simulink model "FAST_11TO14mpers_MPC"  (R2019a)
settings: Solver=FixedStepAuto  StartTime=0.0  StopTime=10  FixedStep=DT  RelTol=1e-3
values from neighbouring files (symbols this model uses):
  Cq = 0.0 0.0 0.0 0.0 0.0 0.0 0.0 0.0 0.0 0.0 0.0 0.0 0.0 0.0 0.0 0.0 0.0 0.0 0.0 0.0 0.0 0.0 0.0 0.0 0.0 0.0 0.0 0.0 0.0 0.0 0.0 0.0 0.0 0.0 0.0 0.0 0.0 0.0 0.0 0.0 0.0 0.0 0.0 0.0 0.0 0.0 0.0 0.0 0.0 0.0 0.0 0.0 0.0 0.0 0.0 0.0 0.0 0.0 0.0 0.0 0.0 0.0 0.0 0.0 0.0 0.0 0.0 0.0 0.0 0.0 0.0 0.0 0.0 0.0 0.0 0.0 0.0 0.0 0.0 0.0 0.0 0.0 0.0 0.0 0.0 0.0 0.0 0.0 0.0 0.0 0.0 0.0 0.0 0.0 0.0 0.0 0.0 0.0 0.0 0.0    [DD_test.sldd]    (also in testOutList.m = saveVarsMat.Cq)
  Drivetrain = struct    [dataDLR.m]
  DT = 0.008    [dataDLR.m]    (also in generateReport.m; initLPVParam.m; initWorkspace.m; runCalculateEvalCriteria.m)
  Lin_points : value not decoded    [DD_test.sldd]
  mu_old = zeros(2*N*nu,1)    [testCtrl.m]
  Ng = 97    [dataDLR.m]    (also in testCtrl.m)
  omegabar = interp1(Lin_points.V,Lin_points.RSpeed,Vbar,'spline')    [testCtrl.m]
  OutList = OutTable.Properties.VariableNames    [initLPVParam.m]    (also in testCtrl.m; testOutList.m = cell(40, 1); testqLPV.m = cell(40, 1))
  tau_g = 0.01    [testCtrl.m]
  U = zeros(2*N,1)    [testCtrl.m]
  Xk07 = kron(ones(N,1),xk07)    [testCtrl.m]
  xk07 = [r7(1), r7(2), zeros(1,5),0]'    [testCtrl.m]
undefined symbols (not defined in the file or in its folder): Rotor_Lambda, Rotor_Lamda, Rotor_Pitch, strmatch
libraries: MdlLib_ProcessOutput x1
settings Model: ExtModeTrigMode=oneshot  ExtModeArmWhenConnect=off  Creator=Hazim Namik  LastModifiedBy=ditt_aj
settings DataIOCC: LimitDataPoints=on  SaveFormat=Array  ReturnWorkspaceOutputs=off
settings OptimizationCC: BlockReduction=off  BooleanDataType=off  LifeSpan=inf
settings DebuggingCC: SaveWithParameterizedLinksMsg=none  UnderspecifiedInitializationDetection=Classic  MergeDetectMultiDrivingBlocksExec=none  SignalResolutionControl=TryResolveAllWithWarning  SFUnexpectedBacktrackingDiag=warning  SFNoUnconditionalDefaultTransitionDiag=warning  SFExecutionAtInitializationDiag=none  ArithmeticOperatorsInVariantConditions=warning
settings HardwareCC: ProdBitPerPointer=32  ProdBitPerSizeT=32  ProdBitPerPtrDiffT=32  ProdLargestAtomicFloat=None  ProdIntDivRoundTo=Undefined  ProdEndianess=Unspecified  ProdWordSize=32  ProdHWDeviceType=32-bit Generic  TargetUnknown=on
settings ModelReferenceCC: PropagateSignalLabelsOutOfModel=off
settings SFSimCC: SimUseLocalCustomCode=off
settings RTWCC: RTWUseLocalCustomCode=off
settings CodeAppCC: StateflowObjectComments=on
settings GRTTargetCC: TargetLangStandard=C89/C90 (ANSI)  GeneratePreprocessorConditionals=Disable all
settings ConfigComp: CovMetricSettings=dw  CovHtmlReporting=on  CovSaveCumulativeToWorkspaceVar=on  CovSaveSingleToWorkspaceVar=on  CovExternalEMLEnable=off

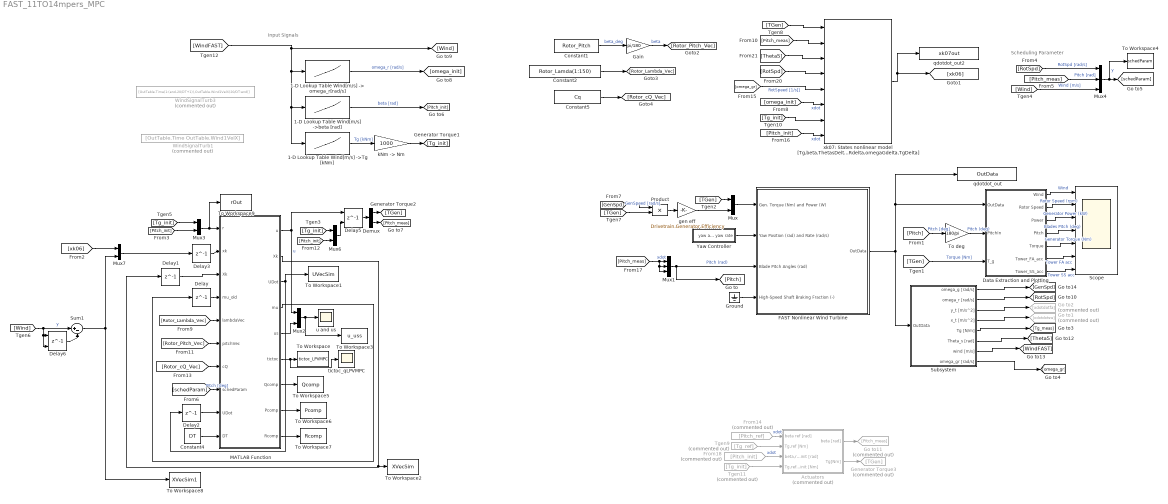
== system FAST_11TO14mpers_MPC ==
  note: Scheduling Parameter
  note: Input Signals
  "1-D Lookup Table Wind[m/s] -> omega_r[rad/s]" : Lookup_n-D  NumberOfTableDimensions=1  BreakpointsForDimension1=Lin_points.V  BreakpointsForDimension2=Rotor_Lambda  Table=Lin_points.RSpeed  InternalRulePriority=Speed  RndMeth=Simplest  InputSameDT=on
  1-D Lookup Table Wind[m/s] ->Tg [kNm] : Lookup_n-D  NumberOfTableDimensions=1  BreakpointsForDimension1=Lin_points.V  BreakpointsForDimension2=Rotor_Lambda  Table=Lin_points.Torque  InternalRulePriority=Speed  RndMeth=Simplest  InputSameDT=on
  1-D Lookup Table Wind[m/s] ->beta [rad] : Lookup_n-D  NumberOfTableDimensions=1  BreakpointsForDimension1=Lin_points.V  BreakpointsForDimension2=Rotor_Lambda  Table=Lin_points.Pitch  InternalRulePriority=Speed  RndMeth=Simplest  InputSameDT=on
  Actuators : Subsystem  Commented=on
  Constant1 : Constant  Value=Rotor_Pitch
  Constant2 : Constant  Value=Rotor_Lamda(1:150)
  Constant4 : Constant  Value=DT
  Constant5 : Constant  Value=Cq
  Data Extraction and Plotting : Subsystem
  Delay : Delay  DelayLength=1  InitialCondition=mu_old
  Delay1 : Delay  DelayLength=1  InitialCondition=Xk07
  Delay2 : Delay  DelayLength=1  InitialCondition=U
  Delay3 : Delay  DelayLength=1  InitialCondition=xk07
  Delay5 : Delay  DelayLength=1  InitialConditionSource=Input port  InitialCondition=[0,omegabar]
      settings: InputPortMap=u0,p4
  Delay6 : Delay  DelayLength=1  InitialConditionSource=Input port  InitialCondition=[0, Lin_points.Torque(1)]
      settings: InputPortMap=u0,p4
  Demux : Demux  Outputs=2
  FAST Nonlinear Wind Turbine : Subsystem  mask(FAST Nonlinear Wind Turbine){}
      mask help: This block contains the FAST S-Function.
      mask init:
      | clear FAST_SFunc
  From14 : From  Commented=on  GotoTag=Pitch_ref
      settings: CloseFcn=tagdialog Close
  From18 : From  Commented=on  GotoTag=Pitch_init
      settings: CloseFcn=tagdialog Close
  Gain : Gain  Gain=pi/180
  Generator Torque3 : Goto  Commented=on  GotoTag=TGen
  Go to1 : Goto  Commented=on  GotoTag=xdotdotsw
  Go to11 : Goto  Commented=on  GotoTag=Pitch_meas
  Go to2 : Goto  Commented=on  GotoTag=xdotdotfa
  Ground : Ground
  MATLAB Function : MATLAB Function  TreatAsAtomicUnit=on
  Mux{,2..3,6..7} (5 alike) : Mux  Inputs=2
  Mux1 : Mux  Inputs=3
  Mux4 : Mux  Inputs=3
  Product : Product  RndMeth=Zero
  Scope : Scope  NumInputPorts=7
      settings: Tag=Scope
  Subsystem : Subsystem
  Sum1 : Sum  Inputs=|+-
  Tgen11 : From  Commented=on  GotoTag=Tg_init
      settings: CloseFcn=tagdialog Close
  Tgen9 : From  Commented=on  GotoTag=Tg_ref
      settings: CloseFcn=tagdialog Close
  To Workspace : ToWorkspace  VariableName=tictoc_LPVMPC  SaveFormat=Timeseries  SampleTime=-1
  To Workspace1 : ToWorkspace  VariableName=UVecSim  SampleTime=-1
  To Workspace2 : ToWorkspace  VariableName=XVecSim  SampleTime=-1
  To Workspace3 : ToWorkspace  VariableName=u_uss  SampleTime=-1
      settings: Save2DSignal=2-D array (concatenate along first dimension)
  To Workspace4 : ToWorkspace  VariableName=schedParam  SampleTime=-1
      settings: Save2DSignal=2-D array (concatenate along first dimension)
  To Workspace5 : ToWorkspace  VariableName=Qcomp  SampleTime=-1
      settings: Save2DSignal=2-D array (concatenate along first dimension)
  To Workspace6 : ToWorkspace  VariableName=Pcomp  SampleTime=-1
      settings: Save2DSignal=2-D array (concatenate along first dimension)
  To Workspace7 : ToWorkspace  VariableName=Rcomp  SampleTime=-1
      settings: Save2DSignal=2-D array (concatenate along first dimension)
  To Workspace8 : ToWorkspace  VariableName=XVecSim1  SampleTime=-1
  To Workspace9 : ToWorkspace  VariableName=rOut  SampleTime=-1
  To deg : Gain  Gain=180/pi
  WindSignalTurb1 : FromWorkspace  Commented=on  VariableName=[OutTable.Time OutTable.Wind1VelX]  SampleTime=DT  OutputAfterFinalValue=Holding final value
  WindSignalTurb3 : FromWorkspace  Commented=on  VariableName=[OutTable.Time(1:(end-20/DT+1)),OutTable.Wind1VelX(20/DT:end)]  SampleTime=DT  OutputAfterFinalValue=Holding final value
  Yaw Controller : Subsystem
  gen eff : Gain  Gain=Drivetrain.Generator.Efficiency
  "kNm -> Nm" : Gain  Gain=1000
  qdotdot_out : ToWorkspace  VariableName=OutData  SampleTime=-1
  qdotdot_out2 : ToWorkspace  VariableName=xk07out  SampleTime=-1
  tictoc_qLPVMPC : Scope
  u and us : Scope
  xk07: States nonlinear model [Tg,beta,ThetasDelta,omegaRdelta,omegaGdelta,TgDelta] : MdlLib_ProcessOutput/xk07: States nonlinear model [Tg,beta,ThetasDelta,omegaRdelta,omegaGdelta,TgDelta]  SystemSampleTime=-1
  wires:
  Mux/1 -> FAST Nonlinear Wind Turbine/1(Gen. Torque (Nm) and Power (W))
  Yaw Controller/1(yaw and yaw rate) -> FAST Nonlinear Wind Turbine/2(Yaw Position (rad) and Rate (rad/s))
  Mux1/1 -> [Pitch], FAST Nonlinear Wind Turbine/3(Blade Pitch Angles (rad))  "Pitch (rad)"
  gen eff/1 -> Mux/2
  Product/1 -> gen eff/1
  Data Extraction and Plotting/3(Power) -> Scope/3  "Generator Power (kW)"
  [Pitch] -> To deg/1  "Pitch [deg]"
  Data Extraction and Plotting/1(Wind) -> Scope/1  "Wind"
  Data Extraction and Plotting/2(Rotor Speed) -> Scope/2  "Rotor Speed (rpm)"
  [TGen] -> Data Extraction and Plotting/3(T_g)  "Torque [Nm]"
  FAST Nonlinear Wind Turbine/1(OutData) -> Subsystem/1(OutData), qdotdot_out/1, Data Extraction and Plotting/1(OutData)
  Data Extraction and Plotting/4(Pitch) -> Scope/4  "Blades Pitch (deg)"
  Data Extraction and Plotting/5(Torque) -> Scope/5  "Generator Torque (Nm)"
  Data Extraction and Plotting/6(Tower_FA_acc) -> Scope/6  "Tower FA acc"
  Data Extraction and Plotting/7(Tower_SS_acc) -> Scope/7  "Tower SS acc"
  Ground/1 -> FAST Nonlinear Wind Turbine/4(High-Speed Shaft Braking Fraction (-))
  [TGen] -> Mux/1
  Subsystem/8(omega_gr [rad/s]) -> [omega_gr]
  Subsystem/3(y_t [m/s^2]) -> Go to2/1
  Subsystem/4(x_t [m/s^2]) -> Go to1/1
  Subsystem/5(Tg [N/m]) -> [Tg_meas]
  [GenSpd] -> Product/1  "GenSpeed [rad/s]"
  [Pitch_meas] -> Mux4/2  "Pitch [rad]"
  [Tg_init] -> xk07: States nonlinear model [Tg,beta,ThetasDelta,omegaRdelta,omegaGdelta,TgDelta]/7
  [Wind] -> Mux4/3  "Wind [m/s]"
  [Pitch_meas] -> xk07: States nonlinear model [Tg,beta,ThetasDelta,omegaRdelta,omegaGdelta,TgDelta]/2
  [RotSpd] -> Mux4/1  "RotSpd [rad/s]"
  [omega_init] -> xk07: States nonlinear model [Tg,beta,ThetasDelta,omegaRdelta,omegaGdelta,TgDelta]/6  "xdot"
  [Pitch_init] -> xk07: States nonlinear model [Tg,beta,ThetasDelta,omegaRdelta,omegaGdelta,TgDelta]/8  "xdot"
  [TGen] -> xk07: States nonlinear model [Tg,beta,ThetasDelta,omegaRdelta,omegaGdelta,TgDelta]/1
  Constant5/1 -> [Rotor_cQ_Vec]
  xk07: States nonlinear model [Tg,beta,ThetasDelta,omegaRdelta,omegaGdelta,TgDelta]/1 -> [xk06], qdotdot_out2/1
  [omega_gr] -> xk07: States nonlinear model [Tg,beta,ThetasDelta,omegaRdelta,omegaGdelta,TgDelta]/5  "RotSpeed [1/s]]"
  [ThetaS] -> xk07: States nonlinear model [Tg,beta,ThetasDelta,omegaRdelta,omegaGdelta,TgDelta]/3
  [RotSpd] -> xk07: States nonlinear model [Tg,beta,ThetasDelta,omegaRdelta,omegaGdelta,TgDelta]/4
  Gain/1 -> [Rotor_Pitch_Vec]  "beta"
  Constant1/1 -> Gain/1  "beta_deg"
  Mux4/1 -> To Workspace4/1, [schedParam]  "y"
  Constant2/1 -> [Rotor_Lambda_Vec]
  [WindFAST] -> "1-D Lookup Table Wind[m/s] -> omega_r[rad/s]"/1, 1-D Lookup Table Wind[m/s] ->beta [rad]/1, 1-D Lookup Table Wind[m/s] ->Tg [kNm]/1, [Wind]
  "1-D Lookup Table Wind[m/s] -> omega_r[rad/s]"/1 -> [omega_init]  "omega_r [rad/s]"
  1-D Lookup Table Wind[m/s] ->Tg [kNm]/1 -> "kNm -> Nm"/1  "Tg [kNm]"
  "kNm -> Nm"/1 -> [Tg_init]
  1-D Lookup Table Wind[m/s] ->beta [rad]/1 -> [Pitch_init]  "beta [rad]"
  Demux/1 -> [TGen]
  MATLAB Function/3(UDot) -> Delay2/1, To Workspace1/1
  Delay6/1 -> Sum1/2
  Delay3/1 -> MATLAB Function/2(xk)
  Delay2/1 -> MATLAB Function/9("UDot ")
  Mux2/1 -> u and us/1, To Workspace3/1
  [Rotor_Lambda_Vec] -> MATLAB Function/5(lambdaVec)
  [Tg_init] -> Mux3/1
  MATLAB Function/7(Qcomp) -> To Workspace5/1
  Constant4/1 -> MATLAB Function/10(DT)
  [Tg_init] -> Mux6/1
  [Pitch_init] -> Mux6/2
  [schedParam] -> MATLAB Function/8(schedParam)  "Pitch [deg]"
  Delay5/1 -> Demux/1
  Mux7/1 -> Delay3/1
  Demux/2 -> [Pitch_meas]
  Mux6/1 -> Delay5/2
  [Wind] -> Delay6/2, Delay6/1, Sum1/1  "y"
  [xk06] -> Mux7/1
  [Rotor_cQ_Vec] -> MATLAB Function/7(cQ)
  Sum1/1 -> To Workspace8/1, Mux7/2
  MATLAB Function/8(Pcomp) -> To Workspace6/1
  MATLAB Function/9(Rcomp) -> To Workspace7/1
  [Rotor_Pitch_Vec] -> MATLAB Function/6(pitchVec)
  Mux3/1 -> To Workspace9/1, MATLAB Function/1(r)
  MATLAB Function/1(u) -> Delay5/1, Mux2/1  "u"
  Delay1/1 -> MATLAB Function/3("Xk ")
  [Pitch_init] -> Mux3/2
  Delay/1 -> MATLAB Function/4(mu_old)
  MATLAB Function/6(tictoc) -> tictoc_qLPVMPC/1, To Workspace/1
  MATLAB Function/2(Xk) -> Delay1/1, To Workspace2/1
  MATLAB Function/4(mu) -> Delay/1
  MATLAB Function/5(us) -> Mux2/2
  [Pitch_meas] -> Mux1/3, Mux1/2, Mux1/1  "xdot"
  Subsystem/2(omega_r [rad/s]) -> [RotSpd]
  Actuators/2(Tg[Nm]) -> Generator Torque3/1
  Tgen9/1 -> Actuators/2(Tg,ref [Nm])
  From14/1 -> Actuators/1(beta ref [rad])  "xdot"
  Actuators/1(beta [rad]) -> Go to11/1
  [TGen] -> Product/2
  Tgen11/1 -> Actuators/4(Tg,ref init [Nm])
  From18/1 -> Actuators/3(beta,ref init [rad])  "xdot"
  Subsystem/6(Theta_s [rad]) -> [ThetaS]
  Subsystem/7(wind [m/s]) -> [WindFAST]
  Subsystem/1(omega_g [rad/s]) -> [GenSpd]
  To deg/1 -> Data Extraction and Plotting/2(PitchIn)  "Pitch (deg)"

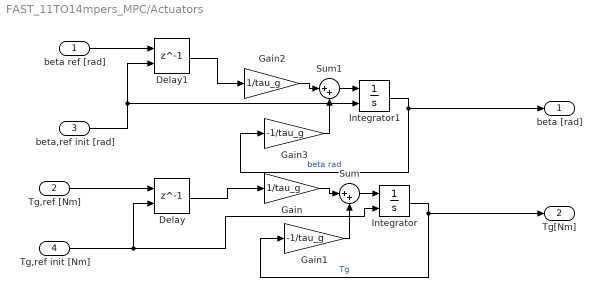
== system FAST_11TO14mpers_MPC/Actuators ==
  beta ref [rad] : Inport
  Tg,ref [Nm] : Inport  Port=2
  beta,ref init [rad] : Inport  Port=3
  Tg,ref init [Nm] : Inport  Port=4
  Delay : Delay  DelayLength=1  InitialConditionSource=Input port
      settings: InputPortMap=u0,p4
  Delay1 : Delay  DelayLength=1  InitialConditionSource=Input port
      settings: InputPortMap=u0,p4
  Gain : Gain  Gain=1/tau_g
  Gain1 : Gain  Gain=-1/tau_g
  Gain2 : Gain  Gain=1/tau_g
  Gain3 : Gain  Gain=-1/tau_g
  Integrator : Integrator  InitialConditionSource=external
  Integrator1 : Integrator  InitialConditionSource=external
  Sum : Sum  Inputs=|++
  Sum1 : Sum  Inputs=|++
  beta [rad] : Outport
  Tg[Nm] : Outport  Port=2
  wires:
  Sum1/1 -> Integrator1/1
  Integrator/1 -> Tg[Nm]/1, Gain1/1  "Tg"
  Tg,ref init [Nm]/1 -> Delay/2, Integrator/2
  Gain3/1 -> Sum1/2
  Gain2/1 -> Sum1/1
  Sum/1 -> Integrator/1
  Gain1/1 -> Sum/2
  Integrator1/1 -> beta [rad]/1, Gain3/1  "beta rad"
  Gain/1 -> Sum/1
  Tg,ref [Nm]/1 -> Delay/1
  Delay/1 -> Gain/1
  beta ref [rad]/1 -> Delay1/1
  Delay1/1 -> Gain2/1
  beta,ref init [rad]/1 -> Integrator1/2, Delay1/2

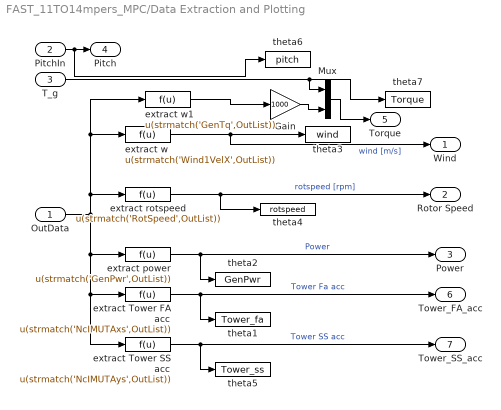
== system FAST_11TO14mpers_MPC/Data Extraction and Plotting ==
  OutData : Inport
  PitchIn : Inport  Port=2
  T_g : Inport  Port=3
  Gain : Gain  Gain=1000
  Mux : Mux  Inputs=2
  extract Tower FA acc : Fcn  Expr=u(strmatch('NcIMUTAxs',OutList))
  extract Tower SS acc : Fcn  Expr=u(strmatch('NcIMUTAys',OutList))
  extract power : Fcn  Expr=u(strmatch('GenPwr',OutList))
  extract rotspeed : Fcn  Expr=u(strmatch('RotSpeed',OutList))
  extract w : Fcn  Expr=u(strmatch('Wind1VelX',OutList))
  extract w1 : Fcn  Expr=u(strmatch('GenTq',OutList))
  theta1 : ToWorkspace  VariableName=Tower_fa  SampleTime=-1
      settings: MaxDataPoints=Inf  Decimation=3
  theta2 : ToWorkspace  VariableName=GenPwr  SampleTime=-1
      settings: MaxDataPoints=Inf  Decimation=3
  theta3 : ToWorkspace  VariableName=wind  SampleTime=-1
      settings: MaxDataPoints=Inf  Decimation=3
  theta4 : ToWorkspace  VariableName=rotspeed  SampleTime=-1
      settings: MaxDataPoints=Inf  Decimation=3
  theta5 : ToWorkspace  VariableName=Tower_ss  SampleTime=-1
      settings: MaxDataPoints=Inf  Decimation=3
  theta6 : ToWorkspace  VariableName=pitch  SampleTime=-1
      settings: MaxDataPoints=Inf  Decimation=3
  theta7 : ToWorkspace  VariableName=Torque  SampleTime=-1
      settings: MaxDataPoints=Inf  Decimation=3
  Wind : Outport
  Rotor Speed : Outport  Port=2
  Power : Outport  Port=3
  Pitch : Outport  Port=4
  Torque : Outport  Port=5
  Tower_FA_acc : Outport  Port=6
  Tower_SS_acc : Outport  Port=7
  wires:
  extract w/1 -> Wind/1, theta3/1  "wind [m/s]"
  extract rotspeed/1 -> theta4/1, Rotor Speed/1  "rotspeed [rpm]"
  extract power/1 -> theta2/1, Power/1  "Power"
  PitchIn/1 -> theta6/1, Pitch/1
  T_g/1 -> Mux/1, theta7/1
  extract Tower FA acc/1 -> theta1/1, Tower_FA_acc/1  "Tower Fa acc"
  OutData/1 -> extract w/1, extract w1/1, extract rotspeed/1, extract Tower SS acc/1, extract Tower FA acc/1, extract power/1
  extract Tower SS acc/1 -> theta5/1, Tower_SS_acc/1  "Tower SS acc"
  extract w1/1 -> Gain/1
  Gain/1 -> Mux/2
  Mux/1 -> Torque/1

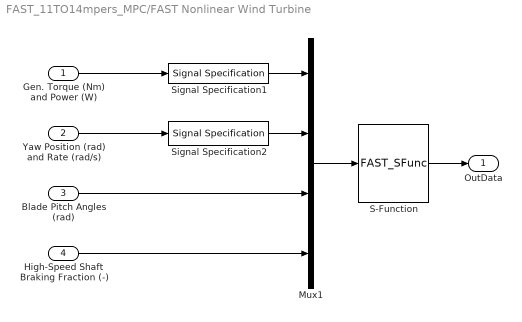
== system FAST_11TO14mpers_MPC/FAST Nonlinear Wind Turbine ==
  Gen. Torque (Nm) and Power (W) : Inport
  Yaw Position (rad) and Rate (rad/s) : Inport  Port=2
  Blade Pitch Angles (rad) : Inport  Port=3
  High-Speed Shaft Braking Fraction (-) : Inport  Port=4
  Mux1 : Mux
  S-Function : S-Function  FunctionName=FAST_SFunc  Parameters=FAST_InputFileName, TMax, 0  SFunctionDeploymentMode=off  EnableBusSupport=off
  Signal Specification1 : SignalSpecification  OutDataTypeStr=double  Dimensions=2
  Signal Specification2 : SignalSpecification  OutDataTypeStr=double  Dimensions=2
  OutData : Outport
  wires:
  Gen. Torque (Nm) and Power (W)/1 -> Signal Specification1/1
  S-Function/1 -> OutData/1
  Mux1/1 -> S-Function/1
  Blade Pitch Angles (rad)/1 -> Mux1/3
  Yaw Position (rad) and Rate (rad/s)/1 -> Signal Specification2/1
  Signal Specification1/1 -> Mux1/1
  Signal Specification2/1 -> Mux1/2
  High-Speed Shaft Braking Fraction (-)/1 -> Mux1/4

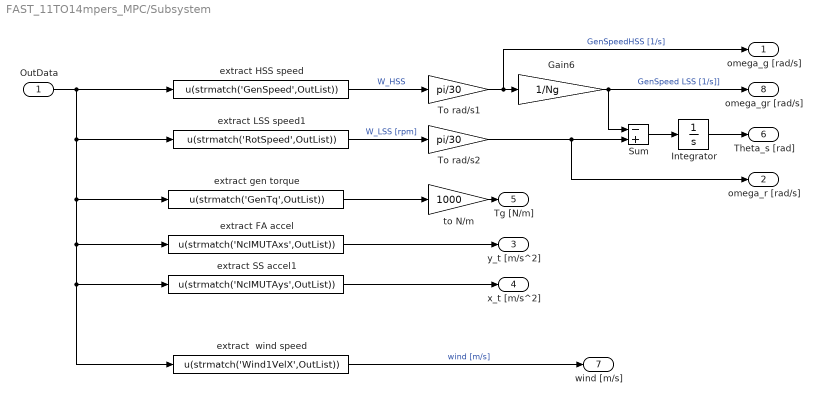
== system FAST_11TO14mpers_MPC/Subsystem ==
  OutData : Inport
  Gain6 : Gain  Gain=1/Ng
  Integrator : Integrator
  Sum : Sum  Inputs=-+
  To rad/s1 : Gain  Gain=pi/30
  To rad/s2 : Gain  Gain=pi/30
  extract  wind speed : Fcn  Expr=u(strmatch('Wind1VelX',OutList))
  extract FA accel : Fcn  Expr=u(strmatch('NcIMUTAxs',OutList))
  extract HSS speed : Fcn  Expr=u(strmatch('GenSpeed',OutList))
  extract LSS speed1 : Fcn  Expr=u(strmatch('RotSpeed',OutList))
  extract SS accel1 : Fcn  Expr=u(strmatch('NcIMUTAys',OutList))
  extract gen torque : Fcn  Expr=u(strmatch('GenTq',OutList))
  to N/m : Gain  Gain=1000
  omega_g [rad/s] : Outport
  omega_r [rad/s] : Outport  Port=2
  y_t [m/s^2] : Outport  Port=3
  x_t [m/s^2] : Outport  Port=4
  Tg [N/m] : Outport  Port=5
  Theta_s [rad] : Outport  Port=6
  wind [m/s] : Outport  Port=7
  omega_gr [rad/s] : Outport  Port=8
  wires:
  to N/m/1 -> Tg [N/m]/1
  OutData/1 -> extract HSS speed/1, extract  wind speed/1, extract SS accel1/1, extract FA accel/1, extract gen torque/1, extract LSS speed1/1
  extract FA accel/1 -> y_t [m/s^2]/1
  extract HSS speed/1 -> To rad/s1/1  "W_HSS"
  extract gen torque/1 -> to N/m/1
  extract SS accel1/1 -> x_t [m/s^2]/1
  To rad/s1/1 -> omega_g [rad/s]/1, Gain6/1  "GenSpeedHSS [1/s]"
  extract LSS speed1/1 -> To rad/s2/1  "W_LSS [rpm]"
  Gain6/1 -> Sum/1, omega_gr [rad/s]/1  "GenSpeed LSS [1/s]]"
  To rad/s2/1 -> Sum/2, omega_r [rad/s]/1
  Sum/1 -> Integrator/1
  Integrator/1 -> Theta_s [rad]/1
  extract  wind speed/1 -> wind [m/s]/1  "wind [m/s]"

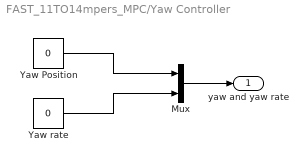
== system FAST_11TO14mpers_MPC/Yaw Controller ==
  Mux : Mux  Inputs=2
  Yaw Position : Constant  Value=0
  Yaw rate : Constant  Value=0
  yaw and yaw rate : Outport
  wires:
  Mux/1 -> yaw and yaw rate/1
  Yaw Position/1 -> Mux/1
  Yaw rate/1 -> Mux/2

== matlab function FAST_11TO14mpers_MPC/MATLAB Function ==
  settings: updateMethod=DISCRETE
  data: r input; u output; xk input; Xk input; mu_old input; lambdaVec input; pitchVec input; cQ input; schedParam input; UDot input; DT input; Xk output; UDot output; mu output; us output; tictoc output; Qcomp output; Pcomp output; Rcomp output
function [u,Xk,UDot,mu,us,tictoc, Qcomp,Pcomp,Rcomp]= qLPVMPC_WECS_beta(r,xk,Xk,mu_old,lambdaVec,pitchVec,cQ,schedParam,UDot,DT)
% MATLAB_Function calculates controller output u. It turns the QP into a 
% linear complementarity problem (LCP) and solves it with Lemke's algorithm.
%
% Inputs: * r: reference
%         * xk: quasiLPV KF state estimates
%         * Xk: Xko(= L*xk+S*U) delayed by one sample timestep
%         * mu_old: mu delayed by one sample timestep
%         * lambdaVec: lambda vector for cQ LUT 
%         * pitchVec: pitch vector for cQ LUT 
%         * cQ: torque coefficients LUT matrix
%         * schedParam: current values [omegaR, beta, V]
%         * U: U (from Xko = L*xk+S*U) delayed by one sample timestep
%
% Outputs: * u: controller output at current time step
%          * Xko: Future state trajectory (L*xk+S*U)
%          * U: Future input trajectory 
%          * mu: Result Lemke's algorithm/LCP: M mu +q >=0, mu>=0, mu'(Mmu+q)=0
%          * us: xuss(end) from xuss = [eye(4)-Ass -Bss;[1 0 0 0] 0]\[Bss*d;1]
%          * tictoc: tic-toc result

% Pablo S.G. Cisneros, Herbert Werner, ICS TUHH

%#codegen
coder.extrinsic('tic');
coder.extrinsic('toc');
tictoc = 0;
tic

%% Init N, Q, R
N = 40;
q_ = [0.1 10^2 0 10^3 10^3 0 0 0]; %[10^4 0.1 1 1 100 0.1 0]; %q_ = [100 1000 1 0.01 0]; 7.351e+02 1.000e+00 1.938e+09 1.625e+08 1.491e+08 1.657e+03
r_ = [0.1 10^2]; %[10^7,0.1];
R_ = kron(eye(N),diag(r_)); %R_ = 1000*eye(N); 
p = 10*q_; %P = 1000*diag(q_);

Ulim = repmat([20000,8 * pi/180]',2*N,1); %rate constraints 

Control_Pitch_Max = 90 /180 * pi;
Control_Pitch_Min = 0 /180 * pi;
Control_Torque_Limit = 47403;
Control_Torque_Min = 200;

% isBetaState = 0;
% nx = 4 + isBetaState; % number states plant: ThetaS,omegaR,omegaG,Tg
% ny = 2 + isBetaState; % number of outputs plant omegaG,Tg
nxA = 8;% nx + ny +clc 1; %number states augmented plant 
nu = 2; % plant inputs: Tg_ref, beta_ref

%% Shift Xk
Xk(1:end-nxA) = Xk(nxA+1:end); 
UDot(1:end-nu) = UDot(nu+1:end);
%Xk(1:nxA)

%% Calculate input u_dot_s = 0  and steady state x = r
us = [0;0]; %xuss(nxA+1:nxA+2); % xuss = [eye(size(Ass))-Ass -Bss;[1 0 0 0] 0] \ [Bss*d;reference];

iterations = 1; % omega_ref(Vest), Tg_ref(Vest)
refVec = zeros(nxA,1);
refVec(1:2) = r;
ref = repmat(refVec,N,1); %ref = kron(ones(N,1),[r; 0; 0; 0;0]);

for i = 1:iterations
    [L,S,H,g] = HSqLd_WT_beta(N,q_,R_,p,xk,Xk,DT,ref,us,lambdaVec,pitchVec,cQ,schedParam,UDot);
    
    %% %%%%%%Turn QP into LCP and solve it%%%%%%%%%
    Ac_ = [-eye(N*nu);eye(N*nu)];
    bc_ = - Ulim;
    Hi = eye(size(H,1))/H;
    M = Ac_*Hi*Ac_';
    q = -Ac_*Hi*g - bc_;
 
    mu = lemke(M,q,mu_old);
 
    UDot = Hi*(Ac_'*mu-g);
    UDot(isnan(UDot)) = 0;
    
    %% %%%%%%%%%%%%%%%%%%%%%%%%%%%%%%%%%%%%%%%%%%%%    
    Xk = L*xk+S*UDot;
end

u =  [ min(max(UDot(1) + Xk(1), Control_Torque_Min),Control_Torque_Limit),... % torque
min( max(UDot(2) + Xk(2), Control_Pitch_Min),Control_Pitch_Max)]'; % pitch

tictoc = toc;

% For debugging
%%%%%%%%%%% Compute Hessian H, derivative g = dJk/dUk %%
% min Jk(Uk) s.t. h1(Uk) = 0, h2(Uk) < 0, at current estimate xl
% <=> min( x'H(xl)x + g(xl)x s.t. dh1(xl)x+h1(xl)=0, dh2(xl)x+h2(xl)< 0
% with 
% Jk = (Lx+SUk-Xss)'Q(Lx+SUk-Xss) +(Uk-Uss)'R(Uk-Uss) + Psi
% dJk/dUk = 2S'Q (Lx+SUk-Xss) + 2R(Uk-Uss) 
diffX = Xk(1:(end - nxA)) - ref(1:(end -nxA));
diffXEnd = Xk((end - nxA +1):end) - ref((end - nxA +1):end);

% Q_ = kron(eye(N-1),diag(q_));
% Qcomp = diffX' * Q_ * diffX;
% Pcomp = diffXEnd' * diag(p)* diffXEnd;
% Rcomp = U' * R_ * U;

diffXMat = sum(reshape(diffX.^2, nxA, N-1),2);
UMat = sum(reshape(UDot.^2, 2, N),2);

Qcomp = diffXMat' .* q_;
Pcomp = (diffXEnd') .^2  .* p;
Rcomp = UMat' .* r_;
